simulink model "GaN_SCRC_Current_Sharing"  (R2022b)
settings: Solver=ode15s  StartTime=0.0  StopTime=8e-6  MaxStep=10e-9  RelTol=1e-9  AbsTol=1e-10
model workspace (MAT data in the model file):
  p.Itotal = 30
  p.VgDUT = 0
  p.VgLS1 = -3
  p.VthDUT = 1.7
  p.VthLS1 = 1.7
  p.Rdut = 0.08
  p.Raux = 0.08
  p.Rshunt = 0.01
  p.Cnode = 2e-10
  p.Rleak = 1000000000
  p.Fdut = 1.7
  p.Faux = 4.7
values from neighbouring files (symbols this model uses):
  p = struct('Itotal',30,'VgDUT',0,'VgLS1',-3,'VthDUT',1.7,'VthLS1',1.7,   'Rdut',.08,'Raux',.08,'Rshunt',.01,'Cnode',200e-12,'Rleak',1e9,'Fdut',1.7,'Faux',4.7)    [build_run_scrc.m]
settings Model: Creator=Greatlovers  LastModifiedBy=Greatlovers

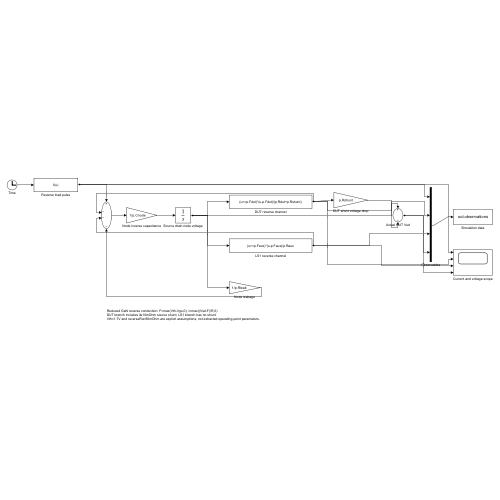
[thumbnail: Simulink's stored preview of the top-level diagram]
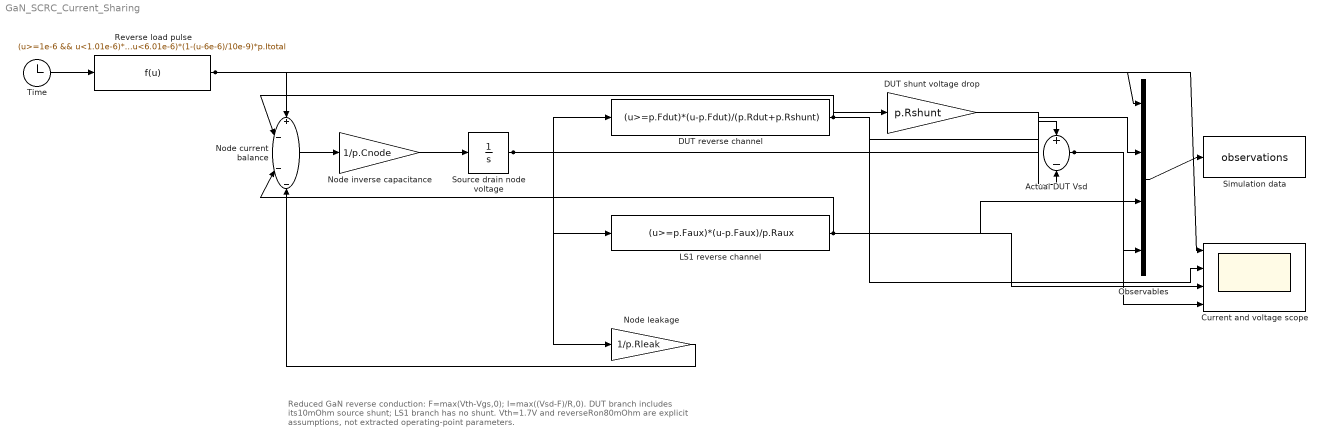
== system GaN_SCRC_Current_Sharing ==
  note: Reduced GaN reverse conduction: F=max(Vth-Vgs,0); I=max((Vsd-F)/R,0).
      | DUT branch includes its10mOhm source shunt; LS1 branch has no shunt.
      | Vth=1.7V and reverseRon80mOhm are explicit assumptions, not extracted operating-point parameters.
  Actual DUT Vsd : Sum  Inputs=+-
  Current and voltage scope : Scope  NumInputPorts=4
  DUT reverse channel : Fcn  Expr=(u>=p.Fdut)*(u-p.Fdut)/(p.Rdut+p.Rshunt)
  DUT shunt voltage drop : Gain  Gain=p.Rshunt
  LS1 reverse channel : Fcn  Expr=(u>=p.Faux)*(u-p.Faux)/p.Raux
  Node current balance : Sum  Inputs=+---
  Node inverse capacitance : Gain  Gain=1/p.Cnode
  Node leakage : Gain  Gain=1/p.Rleak
  Observables : Mux
  Reverse load pulse : Fcn  Expr=(u>=1e-6 && u<1.01e-6)*(u-1e-6)/10e-9*p.Itotal+(u>=1.01e-6 && u<=6e-6)*p.Itotal+(u>6e-6 && u<6.01e-6)*(1-(u-6e-6)/10e-9)*p.Itotal
  Simulation data : ToWorkspace  VariableName=observations  SaveFormat=Timeseries  SampleTime=-1
  Source drain node voltage : Integrator
  Time : Clock
  wires:
  Time/1 -> Reverse load pulse/1
  Reverse load pulse/1 -> Node current balance/1, Observables/1, Current and voltage scope/1
  Node current balance/1 -> Node inverse capacitance/1
  Node inverse capacitance/1 -> Source drain node voltage/1
  Source drain node voltage/1 -> DUT reverse channel/1, LS1 reverse channel/1, Node leakage/1, Actual DUT Vsd/1
  DUT reverse channel/1 -> Node current balance/2, DUT shunt voltage drop/1, Observables/2, Current and voltage scope/2
  LS1 reverse channel/1 -> Node current balance/3, Observables/3, Current and voltage scope/3
  Node leakage/1 -> Node current balance/4
  DUT shunt voltage drop/1 -> Actual DUT Vsd/2
  Actual DUT Vsd/1 -> Observables/4, Current and voltage scope/4
  Observables/1 -> Simulation data/1
